simulink model "trimNonlinearAirframe"  (R2026a)
settings: Solver=ode3  StartTime=0  StopTime=100  FixedStep=Ts  EnableMultiTasking=on
settings Model: Creator=The MathWorks, Inc.  LastModifiedBy=The MathWorks, Inc.
settings DataIOCC: ExternalInput=getinputstruct(op)  InitialState=getstatestruct(op)  SaveFormat=StructureWithTime
settings OptimizationCC: BufferReuse=off
settings DebuggingCC: UnderspecifiedInitializationDetection=Classic
settings HardwareCC: ProdHWDeviceType=32-bit Generic

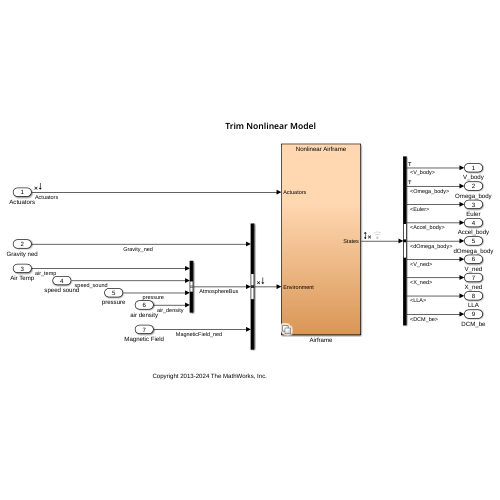
[thumbnail: Simulink's stored preview of the top-level diagram]
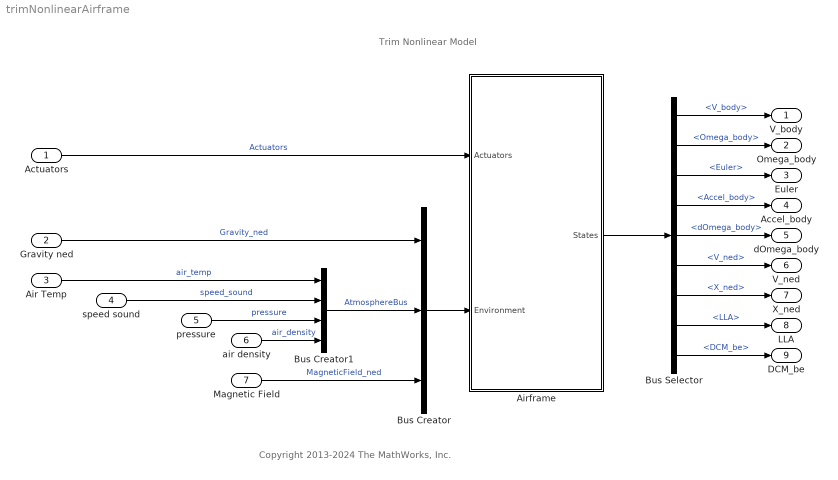
== system trimNonlinearAirframe ==
  note: Trim Nonlinear Model
  note: Copyright 2013-2024 The MathWorks, Inc.
  Actuators : Inport  OutDataTypeStr=double  PortDimensions=[1 4]
  Gravity ned : Inport  Port=2  OutDataTypeStr=double
  Air Temp : Inport  Port=3  OutDataTypeStr=double
  speed sound : Inport  Port=4  OutDataTypeStr=double
  pressure : Inport  Port=5  OutDataTypeStr=double
  air density : Inport  Port=6  OutDataTypeStr=double
  Magnetic Field : Inport  Port=7  OutDataTypeStr=double
  Airframe : Subsystem  Variant=on
  Bus Creator : BusCreator  Inputs=3  OutDataTypeStr=Bus: EnvironmentBus  NonVirtualBus=on
  Bus Creator1 : BusCreator  Inputs=4  OutDataTypeStr=Bus: AtmosphereBus  NonVirtualBus=on
  Bus Selector : BusSelector  OutputSignals=V_body,Omega_body,Euler,Accel_body,dOmega_body,V_ned,X_ned,LLA,DCM_be
  V_body : Outport  VectorParamsAs1DForOutWhenUnconnected=off
  Omega_body : Outport  Port=2  VectorParamsAs1DForOutWhenUnconnected=off
  Euler : Outport  Port=3  VectorParamsAs1DForOutWhenUnconnected=off
  Accel_body : Outport  Port=4  VectorParamsAs1DForOutWhenUnconnected=off
  dOmega_body : Outport  Port=5  VectorParamsAs1DForOutWhenUnconnected=off
  V_ned : Outport  Port=6  VectorParamsAs1DForOutWhenUnconnected=off
  X_ned : Outport  Port=7  VectorParamsAs1DForOutWhenUnconnected=off
  LLA : Outport  Port=8  VectorParamsAs1DForOutWhenUnconnected=off
  DCM_be : Outport  Port=9  VectorParamsAs1DForOutWhenUnconnected=off
  wires:
  Actuators/1 -> Airframe/1(Actuators)  "Actuators"
  Airframe/1(States) -> Bus Selector/1
  Magnetic Field/1 -> Bus Creator/3  "MagneticField_ned"
  Bus Creator1/1 -> Bus Creator/2  "AtmosphereBus"
  air density/1 -> Bus Creator1/4  "air_density"
  pressure/1 -> Bus Creator1/3  "pressure"
  speed sound/1 -> Bus Creator1/2  "speed_sound"
  Air Temp/1 -> Bus Creator1/1  "air_temp"
  Bus Creator/1 -> Airframe/2(Environment)
  Gravity ned/1 -> Bus Creator/1  "Gravity_ned"
  Bus Selector/1 -> V_body/1  "<V_body>"
  Bus Selector/2 -> Omega_body/1  "<Omega_body>"
  Bus Selector/3 -> Euler/1  "<Euler>"
  Bus Selector/4 -> Accel_body/1  "<Accel_body>"
  Bus Selector/5 -> dOmega_body/1  "<dOmega_body>"
  Bus Selector/6 -> V_ned/1  "<V_ned>"
  Bus Selector/7 -> X_ned/1  "<X_ned>"
  Bus Selector/8 -> LLA/1  "<LLA>"
  Bus Selector/9 -> DCM_be/1  "<DCM_be>"

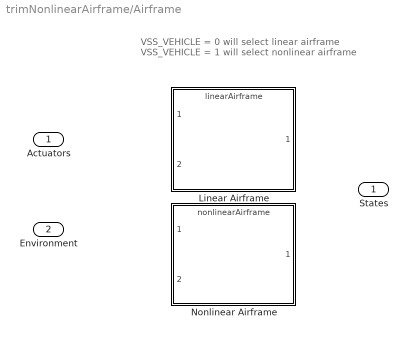
== system trimNonlinearAirframe/Airframe ==
  note: VSS_VEHICLE = 0 will select linear airframe
      | VSS_VEHICLE = 1 will select nonlinear airframe
  Actuators : Inport
  Environment : Inport  Port=2  OutDataTypeStr=Bus: EnvironmentBus
  Linear Airframe : ModelReference  ModelNameDialog=linearAirframe.slx  SimulationMode=Normal  VariantControl=VSS_VEHICLE_LINEAR  ModelReferenceVersion=1.39
  Nonlinear Airframe : ModelReference  ModelNameDialog=nonlinearAirframe.slx  SimulationMode=Normal  VariantControl=VSS_VEHICLE_NONLINEAR  ModelReferenceVersion=1.149
  States : Outport  OutDataTypeStr=Bus: StatesBus  VectorParamsAs1DForOutWhenUnconnected=off
